simulink model "inversor_ex3"  (R2026b)
settings: Solver=VariableStepAuto  StopTime=80  MaxStep=1e-3
InitFcn:
  | run("C:\Users\ArnauCoronado\Documents_local\master\gedit\practica_ppc_Arnau_Coronado_Nadal_gedit\claude_ex3\param_ex3.m")
  | 
  | modelName = bdroot;
  | scopePath = [modelName '/Scope'];
  | 
  | scopeConfig = get_param(scopePath, 'ScopeConfiguration');
  | scopeConfig.Title = scopeTitle;
values from neighbouring files (symbols this model uses):
  P_disp = 2000*ones(1,5)    [param_ex3.m]
  P_init = min(alpha_0*Pn_inv, P_disp)    [param_ex3.m]
  Pn_inv = 2000    [param_ex3.m]
  rate_transition_init_val = alpha_0    (= 0.5)    [param_ex3.m]
  sample_time = 0.2    [param_ex3.m]
  step_time = t_stop    (= 50)    [param_ex3.m]
  t_delay_com = 20e-3    (= 0.02)    [param_ex3.m]
  tau_pv = 0.5    [param_ex3.m]
  transp_delay_init_outp = alpha_0    (= 0.5)    [param_ex3.m]
  transp_delay_pppc_meas = Pppc_0    [param_ex3.m]
libraries: sl_discontinuities x5
settings Model: Creator=arnau.coronado  LastModifiedBy=ArnauCoronado

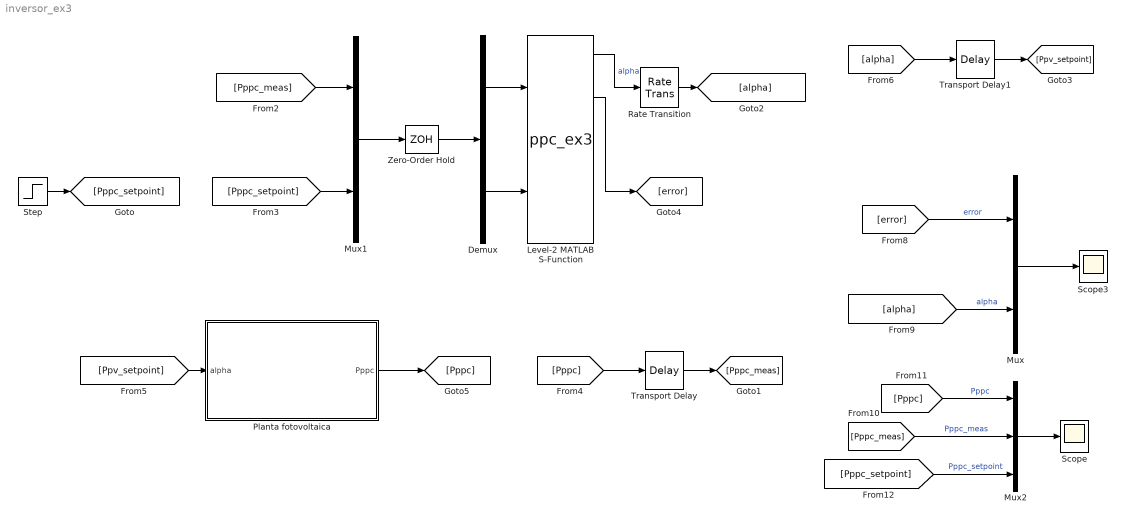
== system inversor_ex3 ==
  Demux : Demux  Outputs=2
  Level-2 MATLAB S-Function : M-S-Function  FunctionName=ppc_ex3  Parameters=sample_time, Ppv_nom, Ki, Kp, Ramp_rate_lim, antiwindup
  Mux : Mux  Inputs=2
  Mux1 : Mux  Inputs=2
  Mux2 : Mux  Inputs=3
  Planta fotovoltaica : Subsystem
  Rate Transition : RateTransition  InitialCondition=rate_transition_init_val
  Scope : Scope
      settings: Title=PPC ej. 3 (caso 1): Kp = 0.5, Ki = 1, anti-windup = 0  ActiveDisplayYMinimum=3021.5643381661353  ActiveDisplayYMaximum=11602.937972149281  YLabel=Power [kW]  DataLoggingVariableName=simout
  Scope3 : Scope
      settings: Title=PPC simulation: Kp = 0.5  ActiveDisplayYMinimum=-3437.3251543825418  ActiveDisplayYMaximum=8648.4698472015352  YLabel=Power [kW]  DataLoggingVariableName=ScopeData4
  Step : Step  Time=step_time  InitialValue=P_tso_ini  FinalValue=P_tso_fin  SampleTime=0
  Transport Delay : TransportDelay  DelayTime=t_delay_com  InitialOutput=transp_delay_pppc_meas
  Transport Delay1 : TransportDelay  DelayTime=t_delay_com  InitialOutput=transp_delay_init_outp
  Zero-Order Hold : ZeroOrderHold  SampleTime=sample_time
  wires:
  Planta fotovoltaica/1(Pppc) -> [Pppc]
  Transport Delay/1 -> [Pppc_meas]
  Step/1 -> [Pppc_setpoint]
  [Pppc_setpoint] -> Mux1/2
  [Pppc_meas] -> Mux1/1
  Mux1/1 -> Zero-Order Hold/1
  Zero-Order Hold/1 -> Demux/1
  Demux/1 -> Level-2 MATLAB S-Function/1
  Demux/2 -> Level-2 MATLAB S-Function/2
  [Pppc] -> Transport Delay/1
  Level-2 MATLAB S-Function/1 -> Rate Transition/1  "alpha"
  Rate Transition/1 -> [alpha]
  [Ppv_setpoint] -> Planta fotovoltaica/1(alpha)
  [alpha] -> Transport Delay1/1
  Transport Delay1/1 -> [Ppv_setpoint]
  Level-2 MATLAB S-Function/2 -> [error]
  [error] -> Mux/1  "error"
  [alpha] -> Mux/2  "alpha"
  [Pppc_meas] -> Mux2/2  "Pppc_meas"
  [Pppc_setpoint] -> Mux2/3  "Pppc_setpoint"
  [Pppc] -> Mux2/1  "Pppc"
  Mux/1 -> Scope3/1
  Mux2/1 -> Scope/1

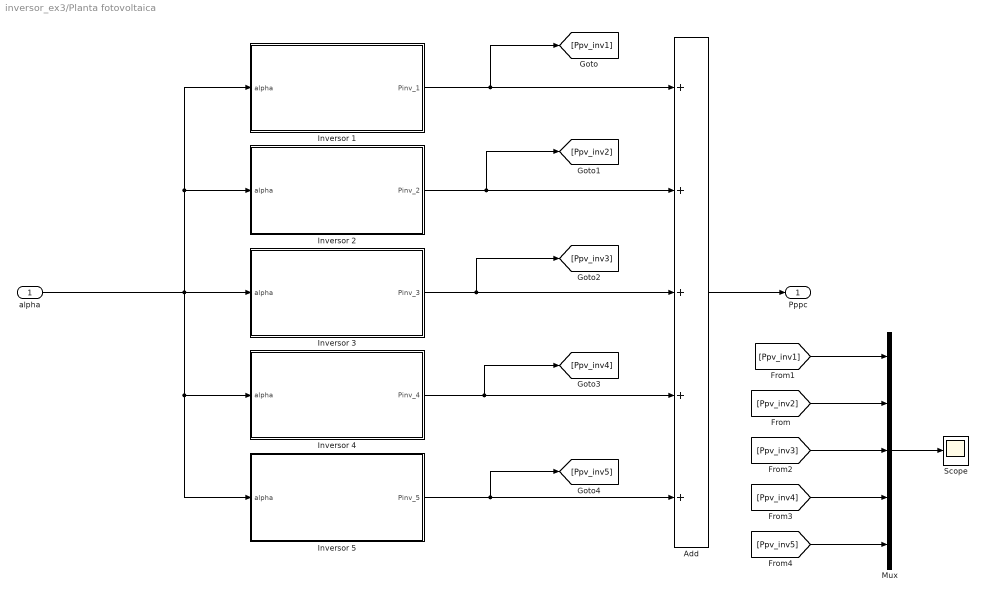
== system inversor_ex3/Planta fotovoltaica ==
  alpha : Inport
  Add : Sum  Inputs=+++++
  Inversor 1 : Subsystem
  Inversor 2 : Subsystem
  Inversor 3 : Subsystem
  Inversor 4 : Subsystem
  Inversor 5 : Subsystem
  Mux : Mux  Inputs=5
  Scope : Scope
      settings: ActiveDisplayYMinimum=-264.44761279829225  ActiveDisplayYMaximum=2491.8023717590063
  Pppc : Outport
  wires:
  Inversor 3/1(Pinv_3) -> Add/3, [Ppv_inv3]
  Inversor 2/1(Pinv_2) -> [Ppv_inv2], Add/2
  Inversor 5/1(Pinv_5) -> Add/5, [Ppv_inv5]
  Inversor 4/1(Pinv_4) -> [Ppv_inv4], Add/4
  Inversor 1/1(Pinv_1) -> Add/1, [Ppv_inv1]
  alpha/1 -> Inversor 4/1(alpha), Inversor 5/1(alpha), Inversor 3/1(alpha), Inversor 2/1(alpha), Inversor 1/1(alpha)
  Add/1 -> Pppc/1
  [Ppv_inv5] -> Mux/5
  [Ppv_inv4] -> Mux/4
  Mux/1 -> Scope/1
  [Ppv_inv3] -> Mux/3
  [Ppv_inv2] -> Mux/2
  [Ppv_inv1] -> Mux/1

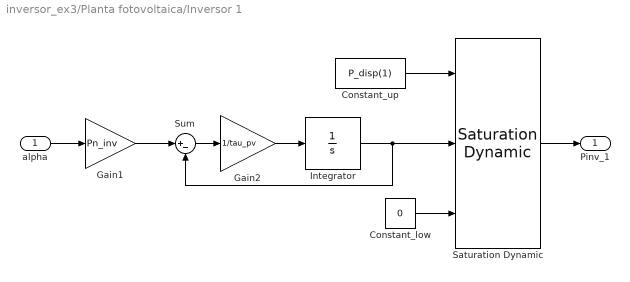
== system inversor_ex3/Planta fotovoltaica/Inversor 1 ==
  alpha : Inport
  Constant_low : Constant  Value=0
  Constant_up : Constant  Value=P_disp(1)
  Gain1 : Gain  Gain=Pn_inv
  Gain2 : Gain  Gain=1/tau_pv
  Integrator : Integrator  InitialCondition=P_init(1)
  Saturation Dynamic : sl_discontinuities/Saturation Dynamic  OutMin=[]  OutMax=[]  OutDataTypeStr=Inherit: Same as second input  OutDataType=fixdt(1, 16)  OutScaling=2^-10  DoSatur=off
      settings: LibrarySourceBlock=|
      | simulink/Discontinuities/Saturation
      | Dynamic
  Sum : Sum  Inputs=|+-
  Pinv_1 : Outport
  wires:
  alpha/1 -> Gain1/1
  Integrator/1 -> Sum/2, Saturation Dynamic/2
  Saturation Dynamic/1 -> Pinv_1/1
  Gain1/1 -> Sum/1
  Sum/1 -> Gain2/1
  Constant_low/1 -> Saturation Dynamic/3
  Gain2/1 -> Integrator/1
  Constant_up/1 -> Saturation Dynamic/1

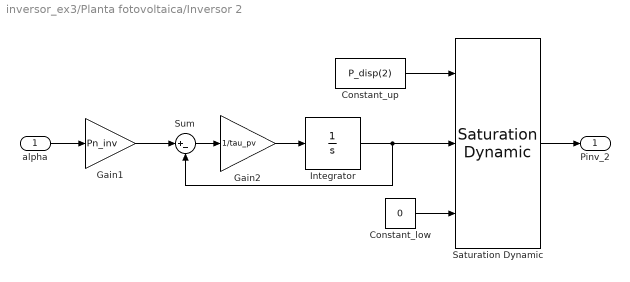
== system inversor_ex3/Planta fotovoltaica/Inversor 2 ==
  alpha : Inport
  Constant_low : Constant  Value=0
  Constant_up : Constant  Value=P_disp(2)
  Gain1 : Gain  Gain=Pn_inv
  Gain2 : Gain  Gain=1/tau_pv
  Integrator : Integrator  InitialCondition=P_init(2)
  Saturation Dynamic : sl_discontinuities/Saturation Dynamic  OutMin=[]  OutMax=[]  OutDataTypeStr=Inherit: Same as second input  OutDataType=fixdt(1, 16)  OutScaling=2^-10  DoSatur=off
      settings: LibrarySourceBlock=|
      | simulink/Discontinuities/Saturation
      | Dynamic
  Sum : Sum  Inputs=|+-
  Pinv_2 : Outport
  wires:
  Constant_up/1 -> Saturation Dynamic/1
  Gain2/1 -> Integrator/1
  Constant_low/1 -> Saturation Dynamic/3
  Sum/1 -> Gain2/1
  Gain1/1 -> Sum/1
  Saturation Dynamic/1 -> Pinv_2/1
  Integrator/1 -> Saturation Dynamic/2, Sum/2
  alpha/1 -> Gain1/1

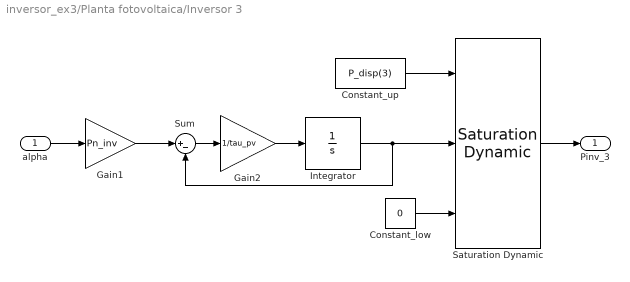
== system inversor_ex3/Planta fotovoltaica/Inversor 3 ==
  alpha : Inport
  Constant_low : Constant  Value=0
  Constant_up : Constant  Value=P_disp(3)
  Gain1 : Gain  Gain=Pn_inv
  Gain2 : Gain  Gain=1/tau_pv
  Integrator : Integrator  InitialCondition=P_init(3)
  Saturation Dynamic : sl_discontinuities/Saturation Dynamic  OutMin=[]  OutMax=[]  OutDataTypeStr=Inherit: Same as second input  OutDataType=fixdt(1, 16)  OutScaling=2^-10  DoSatur=off
      settings: LibrarySourceBlock=|
      | simulink/Discontinuities/Saturation
      | Dynamic
  Sum : Sum  Inputs=|+-
  Pinv_3 : Outport
  wires:
  alpha/1 -> Gain1/1
  Integrator/1 -> Sum/2, Saturation Dynamic/2
  Saturation Dynamic/1 -> Pinv_3/1
  Gain1/1 -> Sum/1
  Sum/1 -> Gain2/1
  Constant_low/1 -> Saturation Dynamic/3
  Gain2/1 -> Integrator/1
  Constant_up/1 -> Saturation Dynamic/1

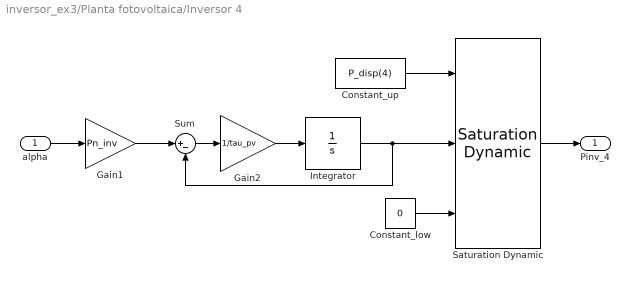
== system inversor_ex3/Planta fotovoltaica/Inversor 4 ==
  alpha : Inport
  Constant_low : Constant  Value=0
  Constant_up : Constant  Value=P_disp(4)
  Gain1 : Gain  Gain=Pn_inv
  Gain2 : Gain  Gain=1/tau_pv
  Integrator : Integrator  InitialCondition=P_init(4)
  Saturation Dynamic : sl_discontinuities/Saturation Dynamic  OutMin=[]  OutMax=[]  OutDataTypeStr=Inherit: Same as second input  OutDataType=fixdt(1, 16)  OutScaling=2^-10  DoSatur=off
      settings: LibrarySourceBlock=|
      | simulink/Discontinuities/Saturation
      | Dynamic
  Sum : Sum  Inputs=|+-
  Pinv_4 : Outport
  wires:
  Constant_up/1 -> Saturation Dynamic/1
  Gain2/1 -> Integrator/1
  Constant_low/1 -> Saturation Dynamic/3
  Sum/1 -> Gain2/1
  Gain1/1 -> Sum/1
  Saturation Dynamic/1 -> Pinv_4/1
  Integrator/1 -> Saturation Dynamic/2, Sum/2
  alpha/1 -> Gain1/1

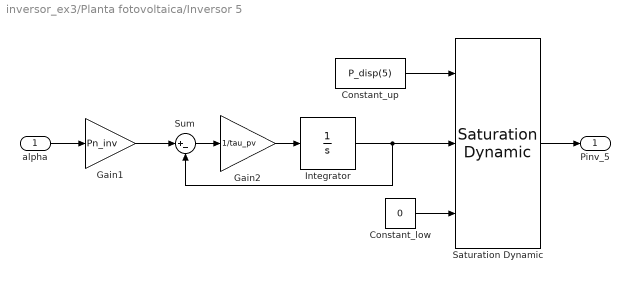
== system inversor_ex3/Planta fotovoltaica/Inversor 5 ==
  alpha : Inport
  Constant_low : Constant  Value=0
  Constant_up : Constant  Value=P_disp(5)
  Gain1 : Gain  Gain=Pn_inv
  Gain2 : Gain  Gain=1/tau_pv
  Integrator : Integrator  InitialCondition=P_init(5)
  Saturation Dynamic : sl_discontinuities/Saturation Dynamic  OutMin=[]  OutMax=[]  OutDataTypeStr=Inherit: Same as second input  OutDataType=fixdt(1, 16)  OutScaling=2^-10  DoSatur=off
      settings: LibrarySourceBlock=|
      | simulink/Discontinuities/Saturation
      | Dynamic
  Sum : Sum  Inputs=|+-
  Pinv_5 : Outport
  wires:
  alpha/1 -> Gain1/1
  Integrator/1 -> Sum/2, Saturation Dynamic/2
  Saturation Dynamic/1 -> Pinv_5/1
  Gain1/1 -> Sum/1
  Sum/1 -> Gain2/1
  Constant_low/1 -> Saturation Dynamic/3
  Gain2/1 -> Integrator/1
  Constant_up/1 -> Saturation Dynamic/1
